simulink model "vsc_hvdc_hysteresis_control"  (R2024b)
settings: Solver=VariableStepAuto  StartTime=0.0  StopTime=0.1  RelTol=1e-3
libraries: spsDCVoltageSourceLib x1, spsGroundLib x1, spsPLL3phLib x1, spsPower3phInstantaneousLib x1, spsThreePhaseVIMeasurementLib x1, spsThreePhaseSeriesRLCBranchLib x1, spsThreePhaseSourceLib x1, spsUniversalBridgeLib x1, spsVoltageMeasurementLib x1, sps_lib x1
settings Model: Creator=Eng.Abd-Elrhman Saad  LastModifiedBy=Eng.Abd-Elrhman Saad

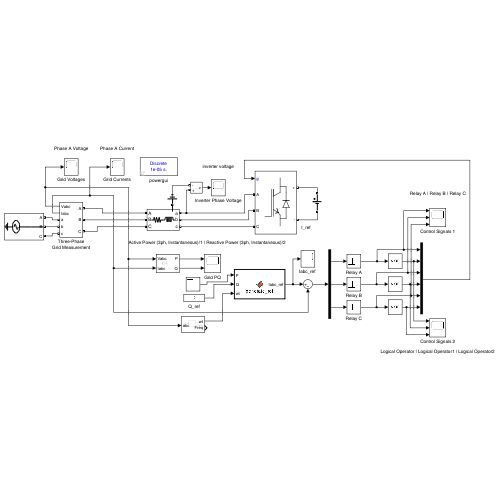
[thumbnail: Simulink's stored preview of the top-level diagram]
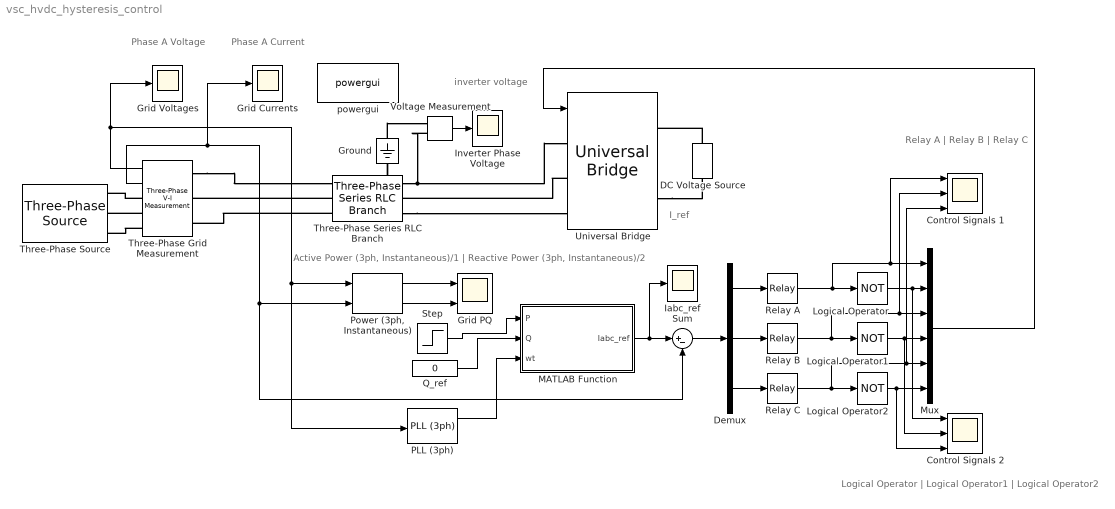
== system vsc_hvdc_hysteresis_control ==
  note: Relay A | Relay B | Relay C
  note: Logical Operator | Logical Operator1 | Logical Operator2
  note: Phase A Current
  note: Active Power (3ph, Instantaneous)/1 | Reactive Power (3ph, Instantaneous)/2
  note: Phase A Voltage
  note: I_ref
  note: inverter voltage
  Control Signals 1 : Scope  NumInputPorts=3
  Control Signals 2 : Scope  NumInputPorts=3
  DC Voltage Source : spsDCVoltageSourceLib/DC Voltage Source  Amplitude=200000  Measurements=None
  Demux : Demux  Outputs=3
  Grid Currents : Scope
  Grid PQ : Scope  NumInputPorts=2
  Grid Voltages : Scope
  Ground : spsGroundLib/Ground  LConnTagsString=a
  "Iabc_ref " : Scope
  Inverter Phase Voltage : Scope
  Logical Operator : Logic  Operator=NOT  AllPortsSameDT=off
  Logical Operator1 : Logic  Operator=NOT  AllPortsSameDT=off
  Logical Operator2 : Logic  Operator=NOT  AllPortsSameDT=off
  MATLAB Function : MATLAB Function  TreatAsAtomicUnit=on
  Mux : Mux  Inputs=6
  PLL (3ph) : spsPLL3phLib/PLL (3ph)  Fmin=45  Par_Init=[0, 50]  ParK=[180, 3200, 1]  TcD=1e-4  MaxRateChangeFreq=12  FilterCutOffFreq=25  Ts=0  AGC=on
  "Power (3ph, Instantaneous)" : spsPower3phInstantaneousLib/Power (3ph, Instantaneous)
  Q_ref : Constant  Value=0
  Relay A : Relay  OnSwitchValue=50  OffSwitchValue=-50  OutDataTypeStr=boolean
  Relay B : Relay  OnSwitchValue=50  OffSwitchValue=-50  OutDataTypeStr=boolean
  Relay C : Relay  OnSwitchValue=50  OffSwitchValue=-50  OutDataTypeStr=boolean
  Step : Step  Time=0.05  Before=405e6  After=-405e6  SampleTime=0
  Sum : Sum  Inputs=|+-
  Three-Phase Grid Measurement : spsThreePhaseVIMeasurementLib/Three-Phase V-I Measurement  VoltageMeasurement=phase-to-ground  SetLabelV=off  LabelV=Vabc  Vpu=off  VpuLL=off  CurrentMeasurement=yes  SetLabelI=off  LabelI=Iabc  Ipu=off  Pbase=100e6  Vbase=500e3  OutputType=Complex  PhasorSimulation=off  PSBequivalent=0
  Three-Phase Series RLC Branch : spsThreePhaseSeriesRLCBranchLib/Three-Phase Series RLC Branch  LConnTagsString=A|B|C  RConnTagsString=A|B|C  BranchType=RL  Resistance=0.5  Inductance=5/(2*pi*50)  Capacitance=1e-6  Measurements=None
  Three-Phase Source : spsThreePhaseSourceLib/Three-Phase Source  InternalConnection=Yg  VoltagePhases=off  Voltage=90e3 * sqrt(1.5)  PhaseAngle=0  Voltage_phases=[25e3 25e3 25e3]/sqrt(3)  PhaseAngles_phases=[0 -120 +120]  Frequency=50  NonIdealSource=off  SpecifyImpedance=off  Resistance=0.8929  Inductance=16.58e-3  ShortCircuitLevel=100e6  BaseVoltage=25e3  XRratio=7  BusType=swing  Pref=10e3  Qref=0  Prefabc=[10e3, 10e3, 10e3]  Qrefabc=[0, 0, 0]  Qmin=-inf  Qmax=inf
  Universal Bridge : spsUniversalBridgeLib/Universal Bridge  Arms=3  SnubberResistance=1e5  SnubberCapacitance=inf  Device=IGBT / Diodes  Ron=1e-3  Lon=0  ForwardVoltages="[  0  0  ]"  ForwardVoltage=0  GTOparameters=[ 10e-6 , 20e-6 ]  IGBTparameters=[ 1e-6 , 2e-6 ]  Measurements=None  Measurements_2=None  converterType=Rectifier
  Voltage Measurement : spsVoltageMeasurementLib/Voltage Measurement  PhasorSimulation=off  OutputType=Complex  PSBequivalent=0
  powergui : sps_lib/powergui  Priority=1  SimulationMode=Discrete  SampleTime=1e-5  frequency=60  Iterations=50  frequencyindice=50  Pbase=100e6  ErrMax=1e-4  UnitsV=kV  UnitsW=MW  buscounter=0  FunctionMessages=off  echomessages=off  EnableUseOfTLC=off  CurrentSourceSwitches=off  DisableSnubberDevices=off  DisableRonSwitches=off  DisableVfSwitches=off  DisplayEquations=off  AutomaticDiscreteSolvers=off  SolverType=Tustin/Backward Euler (TBE)  Interpol=off  ExternalGateDelay=off  methode=off  Ts=100  x0status=blocks  SPID=on  SwTol=0  HookPort=off  NonlinearTolerance=1e-4  nMaxIteration=100  ContinueOnMaxIteration=off  RestoreLinks=warning  ResistiveCurrentMeasurement=off  Frange=[0:2:500]  Ylog=off  Xlog=on  ShowGrid=off  save=off  variable=ZData  structure=0  ZoomFFT=off  StartTime=0.0  cycles=1  DisplayStyle=1  fundamental=60  FreqAxis=off  MaxFrequency=1000  frequencyindicesteady=1  RmsSteady=1  display=off
  wires:
  Three-Phase Grid Measurement/1 -> Grid Voltages/1, "Power (3ph, Instantaneous)"/1, PLL (3ph)/1
  Three-Phase Grid Measurement/2 -> "Power (3ph, Instantaneous)"/2, Sum/2, Grid Currents/1
  PLL (3ph)/2 -> MATLAB Function/3(wt)
  MATLAB Function/1(Iabc_ref) -> Sum/1, "Iabc_ref "/1
  Sum/1 -> Demux/1
  Demux/3 -> Relay C/1
  Demux/2 -> Relay B/1
  Demux/1 -> Relay A/1
  Mux/1 -> Universal Bridge/1
  Q_ref/1 -> MATLAB Function/2(Q)
  "Power (3ph, Instantaneous)"/2 -> Grid PQ/2
  "Power (3ph, Instantaneous)"/1 -> Grid PQ/1
  Voltage Measurement/1 -> Inverter Phase Voltage/1
  Relay A/1 -> Control Signals 1/1, Mux/1, Logical Operator/1
  Relay B/1 -> Mux/3, Control Signals 1/2, Logical Operator1/1
  Relay C/1 -> Mux/5, Control Signals 1/3, Logical Operator2/1
  Logical Operator/1 -> Mux/2, Control Signals 2/1
  Logical Operator1/1 -> Mux/4, Control Signals 2/2
  Logical Operator2/1 -> Mux/6, Control Signals 2/3
  Step/1 -> MATLAB Function/1(P)
  connections:
  Universal Bridge/RConn2 -- DC Voltage Source/LConn1
  Three-Phase Series RLC Branch/RConn1 -- Voltage Measurement/LConn1 -- Universal Bridge/LConn1
  Three-Phase Series RLC Branch/RConn3 -- Universal Bridge/LConn3
  Universal Bridge/LConn2 -- Three-Phase Series RLC Branch/RConn2
  Three-Phase Grid Measurement/RConn2 -- Three-Phase Source/RConn2
  Three-Phase Grid Measurement/RConn1 -- Three-Phase Source/RConn1
  Three-Phase Grid Measurement/RConn3 -- Three-Phase Source/RConn3
  Three-Phase Grid Measurement/LConn1 -- Three-Phase Series RLC Branch/LConn1
  Three-Phase Series RLC Branch/LConn2 -- Three-Phase Grid Measurement/LConn2
  Three-Phase Series RLC Branch/LConn3 -- Three-Phase Grid Measurement/LConn3
  DC Voltage Source/RConn1 -- Universal Bridge/RConn1
  Ground/LConn1 -- Voltage Measurement/LConn2

== matlab function vsc_hvdc_hysteresis_control/MATLAB Function ==
  data: P input; Iabc_ref output; Q input; wt input
function Iabc_ref = generate_ref(P, Q, wt)
    Vm = 90000; % Peak phase voltage from the sheet
    
    % Calculate peak current
    S = sqrt(P^2 + Q^2);
    Im = (2/3) * (S / Vm);
    
    % Calculate power factor angle
    phi = atan2(Q, P);
    
    % Generate 3-phase reference currents
    Ia = Im * sin(wt - phi);
    Ib = Im * sin(wt - 2*pi/3 - phi);
    Ic = Im * sin(wt + 2*pi/3 - phi);
    
    Iabc_ref = [Ia; Ib; Ic];
end
